simulink model "system_model_NMPC"  (R2025b)
settings: Solver=ode45  StartTime=0.0  StopTime=40000  MaxStep=1.5  RelTol=1e-9
values from neighbouring files (symbols this model uses):
  a_leader = 6786 *10^3    (= 6786000)    [main_setup.m]
  delta_a_ref = 0    [ControllerPerformance.m]    (also in evaluate_orbit_control.m = expandReference(delta_a_ref, n, 'delta_a_ref'); main_setup.m)
  delta_lambda_ref = 20/a_leader    [ControllerPerformance.m]    (also in evaluate_orbit_control.m = expandReference(delta_lambda_ref, n, 'delta_lambda_ref'); main_setup.m = 2.94724432655e-06)
  earth_radi = 6371*10^3    (= 6371000)    [main_setup.m]
  J2 = 1.08263e-3    (= 0.00108263)    [nmpc_orbit_state.m]
  J_2 = 1.08263 * 10^(-3)    (= 0.00108263)    [main_setup.m]
  Kd_follower = 2*zeta_follower*wn_follower *                [Jx_follower ... (first row only)    [ATTITUDE_INITIALS.m]
  Kd_leader = 2*zeta_leader*wn_leader *              [Jx_leader ... (first row only)    [ATTITUDE_INITIALS.m]
  Kp_follower = [Jx_follower ... (first row only)    [ATTITUDE_INITIALS.m]
  Kp_leader = [Jx_leader ... (first row only)    [ATTITUDE_INITIALS.m]
  m_f = 2    [main_setup.m]
  m_l = 2    [main_setup.m]
  Mmax_follower = [3.2e-3 ... (first row only)    [ATTITUDE_INITIALS.m]
  Mmax_leader = [3.2e-3 ... (first row only)    [ATTITUDE_INITIALS.m]
  mu = G*earth_mass    (= 398589196000000)    [main_setup.m]    (also in nmpc_orbit_state.m)
  rho_leader = mean_rho_500km    (= 7.3e-13)    [main_setup.m]
undefined symbols (not defined in the file or in its folder): beta0_sdre, beta_max_sdre, beta_min_sdre, Q_sdre, R_sdre
libraries: mpclib x1
(part 1 of 3)
settings Model: Creator=andrefan  LastModifiedBy=Lenovo
settings DataIOCC: FinalStateName=system_modelSimState  InitialState=system_modelSimState  SaveFinalState=on  SaveOperatingPoint=on
settings OptimizationCC: DefaultParameterBehavior=Inlined  UseDivisionForNetSlopeComputation=on  GainParamInheritBuiltInType=on  UseFloatMulNetSlope=on  InlineInvariantSignals=on  FunctionInliningControlUserFunctions=Never  FunctionInliningControlMWFunctions=Readability  FunctionInliningControlMWUserFunctions=Never  PassReuseOutputArgsAs=Individual arguments  ZeroExternalMemoryAtStartup=off  ZeroInternalMemoryAtStartup=off  NoFixptDivByZeroProtection=on  EfficientFloat2IntCast=on  LifeSpan=1  OptimizeBlockOrder=speed  DifferentSizesBufferReuse=on  EfficientTunableParamExpr=on
settings DebuggingCC: ParameterTunabilityLossMsg=error
settings HardwareCC: ProdLongLongMode=on
settings SFSimCC: MATLABDynamicMemAlloc=off
settings RTWCC: SystemTargetFile=ert.tlc  GenCodeOnly=on  TemplateMakefile=ert_default_tmf  BuildConfiguration=Debug  GPUComputeCapability=3.5  Description=Embedded Coder
settings CodeAppCC: ForceParamTrailComments=on  IgnoreCustomStorageClasses=off  OperatorAnnotations=on  SimulinkDataObjDesc=on  SFDataObjDesc=on  CustomSymbolStrGlobalVar=rt$N$M  CustomSymbolStrType=$N$M  CustomSymbolStrFcn=$N$M$F  CustomSymbolStrMacro=$N$M  InsertBlockDesc=on
settings ERTTargetCC: ERTCustomFileTemplate=example_file_process.tlc  ERTFilePackagingFormat=CompactWithDataFile  TargetLangStandard=C99 (ISO)  GenerateSampleERTMain=on  IncludeMdlTerminateFcn=off  CombineSignalStateStructs=on  SupportAbsoluteTime=off  SupportComplex=off  SupportContinuousTime=on  SupportNonInlinedSFcns=on

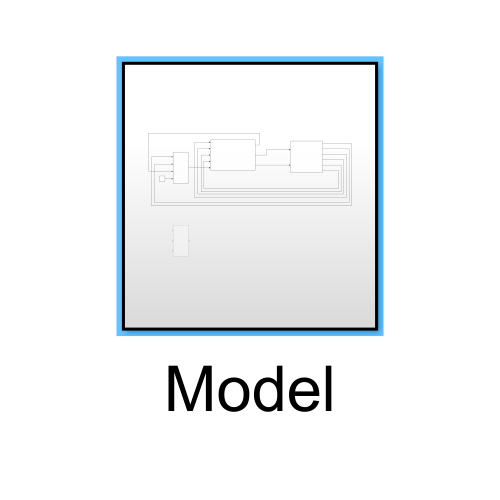
[thumbnail: Simulink's stored preview of the top-level diagram]
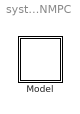
== system system_model_NMPC ==
  Model : Subsystem

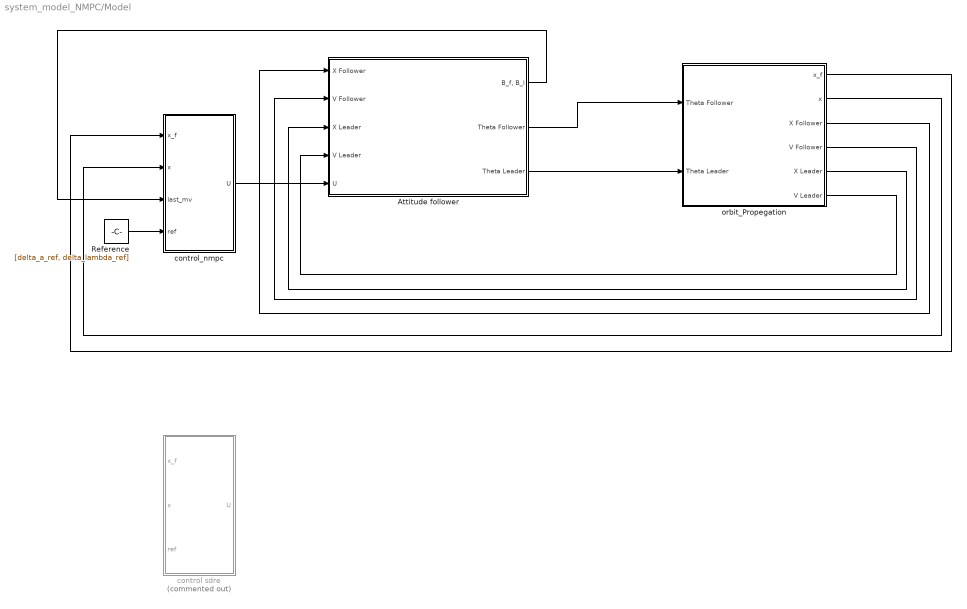
== system system_model_NMPC/Model ==
  "Attitude follower " : Subsystem
  Reference : Constant  Value=[delta_a_ref, delta_lambda_ref]
  control sdre : Subsystem  Commented=on
  control_nmpc : Subsystem
  orbit_Propegation : Subsystem
  wires:
  orbit_Propegation/1(x_f) -> control_nmpc/1(x_f)
  orbit_Propegation/2(x) -> control_nmpc/2(x)
  Reference/1 -> control_nmpc/4(ref)
  orbit_Propegation/3(X Follower) -> "Attitude follower "/1(X Follower)
  orbit_Propegation/4(V Follower) -> "Attitude follower "/2(V Follower)
  orbit_Propegation/5(X Leader) -> "Attitude follower "/3(X Leader)
  orbit_Propegation/6(V Leader) -> "Attitude follower "/4(V Leader)
  "Attitude follower "/2(Theta Follower) -> orbit_Propegation/1(Theta Follower)
  "Attitude follower "/3(Theta Leader) -> orbit_Propegation/2(Theta Leader)
  control_nmpc/1(U) -> "Attitude follower "/5(U)
  "Attitude follower "/1("B_f, B_l") -> control_nmpc/3(last_mv)

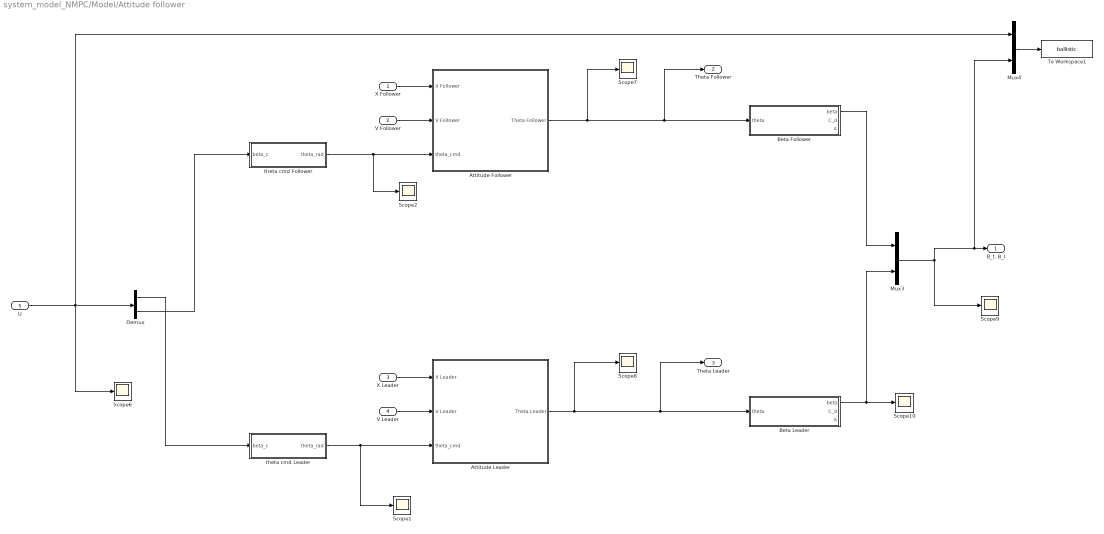
== system system_model_NMPC/Model/Attitude follower  ==
  X Follower : Inport
  V Follower : Inport  Port=2
  X Leader : Inport  Port=3
  V Leader : Inport  Port=4
  U : Inport  Port=5
  Attitude Follower : Subsystem
  Attitude Leader : Subsystem
  Beta Follower : MATLAB Function  TreatAsAtomicUnit=on
  Beta Leader : MATLAB Function  TreatAsAtomicUnit=on
  Demux : Demux  Outputs=2
  Mux3 : Mux  Inputs=2
  Mux4 : Mux  Inputs=2
  Scope{1..2,6..10} (7 alike) : Scope
      Scope1 settings: ActiveDisplayYMinimum=-0.045913062602693733  ActiveDisplayYMaximum=1.4555864748650962  DataLoggingVariableName=ScopeData43
      Scope10 settings: ActiveDisplayYMinimum=-0.0089508661365174519  ActiveDisplayYMaximum=0.27107619634307356  DataLoggingVariableName=ScopeData40
      Scope2 settings: ActiveDisplayYMinimum=-0.18250820694100406  ActiveDisplayYMaximum=1.6425738624690367
      Scope6 settings: ActiveDisplayYMinimum=0.0048104776645491263  ActiveDisplayYMaximum=0.08683060912495788  DataLoggingVariableName=ScopeData41
      Scope7 settings: ActiveDisplayYMinimum=-0.14955674609276967  ActiveDisplayYMaximum=1.3420939307289279  DataLoggingVariableName=ScopeData42
      Scope8 settings: ActiveDisplayYMinimum=-4.5513250658678969E-5  ActiveDisplayYMaximum=0.0004096192559281108  DataLoggingVariableName=ScopeData43
      Scope9 settings: ActiveDisplayYMinimum=-0.051056264121872613  ActiveDisplayYMaximum=0.257673572261877  DataLoggingVariableName=ScopeData38
  To Workspace1 : ToWorkspace  VariableName=ballistic  SaveFormat=Timeseries  SampleTime=-1
  theta cmd Follower : MATLAB Function  TreatAsAtomicUnit=on
  theta cmd Leader : MATLAB Function  TreatAsAtomicUnit=on
  "B_f, B_l" : Outport
  Theta Follower : Outport  Port=2
  Theta Leader : Outport  Port=3
  wires:
  X Follower/1 -> Attitude Follower/1(X Follower)
  V Follower/1 -> Attitude Follower/2(V Follower)
  X Leader/1 -> Attitude Leader/1(X Leader)
  V Leader/1 -> Attitude Leader/2(V Leader)
  theta cmd Leader/1(theta_rad) -> Scope1/1, Attitude Leader/3(theta_cmd)
  theta cmd Follower/1(theta_rad) -> Scope2/1, Attitude Follower/3(theta_cmd)
  Attitude Follower/1(Theta Follower) -> Theta Follower/1, Beta Follower/1(theta), Scope7/1
  Attitude Leader/1(Theta Leader) -> Scope8/1, Theta Leader/1, Beta Leader/1(theta)
  Beta Leader/1(beta) -> Mux3/2, Scope10/1
  Mux3/1 -> Scope9/1, Mux4/2, "B_f, B_l"/1
  Beta Follower/1(beta) -> Mux3/1
  Mux4/1 -> To Workspace1/1
  U/1 -> Mux4/1, Scope6/1, Demux/1
  Demux/1 -> theta cmd Leader/1(beta_c)
  Demux/2 -> theta cmd Follower/1(beta_c)

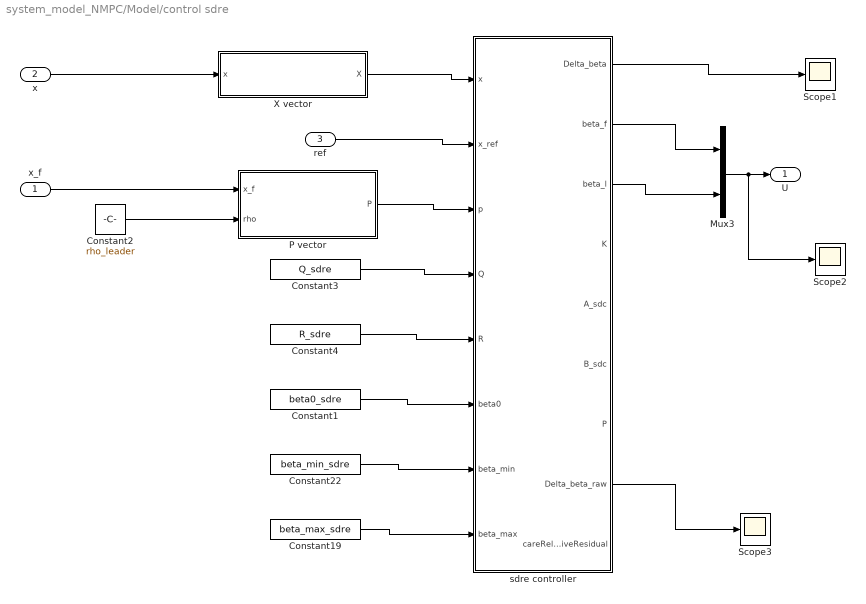
== system system_model_NMPC/Model/control sdre ==
  x_f : Inport
  x : Inport  Port=2
  ref : Inport  Port=3
  Constant1 : Constant  Value=beta0_sdre
  Constant19 : Constant  Value=beta_max_sdre
  Constant2 : Constant  Value=rho_leader
  Constant22 : Constant  Value=beta_min_sdre
  Constant3 : Constant  Value=Q_sdre
  Constant4 : Constant  Value=R_sdre
  Mux3 : Mux  Inputs=2
  P vector : MATLAB Function  TreatAsAtomicUnit=on
  Scope1 : Scope
      settings: ActiveDisplayYMinimum=-0.0032921639354863029  ActiveDisplayYMaximum=-0.0014749131731903909  DataLoggingVariableName=ScopeData14
  Scope2 : Scope
      settings: ActiveDisplayYMinimum=0.0407755493500229  ActiveDisplayYMaximum=0.054229976864297966  DataLoggingVariableName=ScopeData3
  Scope3 : Scope
      settings: ActiveDisplayYMinimum=0.033685370004966811  ActiveDisplayYMaximum=0.084038625678476891  DataLoggingVariableName=ScopeData5
  X vector : MATLAB Function  TreatAsAtomicUnit=on
  sdre controller : MATLAB Function  TreatAsAtomicUnit=on
  U : Outport
  wires:
  P vector/1(P) -> sdre controller/3(p)
  Constant2/1 -> P vector/2(rho)
  x_f/1 -> P vector/1(x_f)
  x/1 -> X vector/1(x)
  X vector/1(X) -> sdre controller/1(x)
  Constant19/1 -> sdre controller/8(beta_max)
  Constant22/1 -> sdre controller/7(beta_min)
  Constant1/1 -> sdre controller/6(beta0)
  Constant3/1 -> sdre controller/4(Q)
  sdre controller/2(beta_f) -> Mux3/1
  sdre controller/3(beta_l) -> Mux3/2
  Mux3/1 -> U/1, Scope2/1
  ref/1 -> sdre controller/2(x_ref)
  sdre controller/1(Delta_beta) -> Scope1/1
  sdre controller/8(Delta_beta_raw) -> Scope3/1
  Constant4/1 -> sdre controller/5(R)

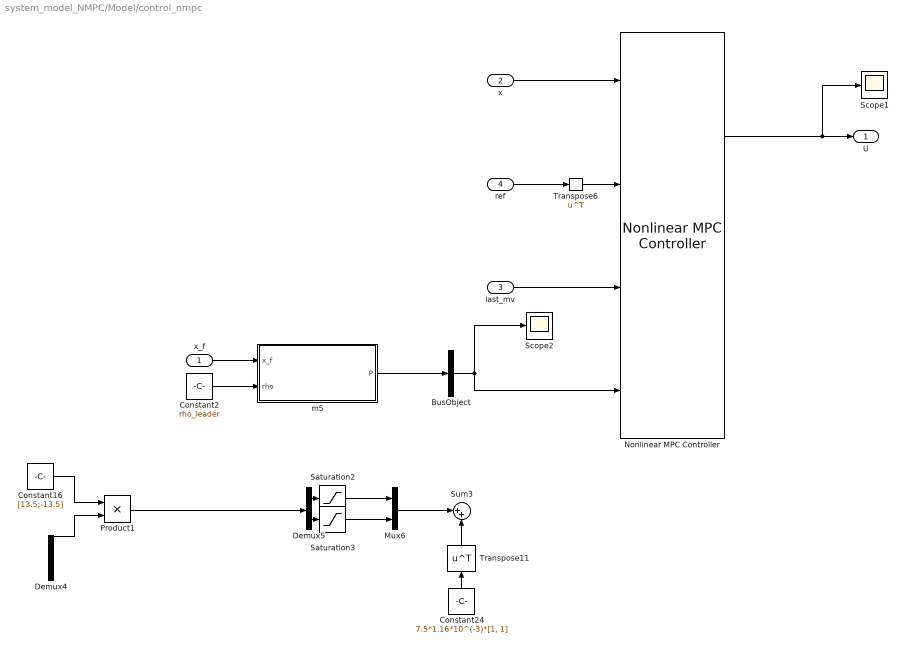
== system system_model_NMPC/Model/control_nmpc ==
  x_f : Inport
  x : Inport  Port=2
  last_mv : Inport  Port=3
  ref : Inport  Port=4
  BusObject : BusCreator  Inputs=1  OutDataTypeStr=Bus: BusObject  NonVirtualBus=on
      settings: InheritFromInputs=off
  Constant16 : Constant  Value=[13.5;-13.5]
  Constant2 : Constant  Value=rho_leader
  Constant24 : Constant  Value=7.5*1.16*10^(-3)*[1, 1]
  Demux4 : Demux  Outputs=6
  Demux5 : Demux  Outputs=2
  Mux6 : Mux  Inputs=2
  Nonlinear MPC Controller : mpclib/Nonlinear MPC Controller  nlmpcobj=nlobj  UseObjectTs=on  TsControl=20  UseMEX=off  md_enabled=off  mvtarget_enabled=off  param_enabled=on  cost_enabled=on  mvseq_enabled=off  stateseq_enabled=off  ovseq_enabled=off  slack_enabled=off  status_enabled=off  ov_min=off  ov_max=off  mv_min=off  mv_max=off  mvrate_min=off  mvrate_max=off  state_min=off  state_max=off  ov_weight=off  mv_weight=off  mvrate_weight=off  ecr_weight=off  nlp_initialize=off
  Product1 : Product
  Saturation2 : Saturate  UpperLimit=inf  LowerLimit=0.000348
  Saturation3 : Saturate  UpperLimit=inf  LowerLimit=0.000348
  Scope1 : Scope
      settings: ActiveDisplayYMinimum=0.00481047337988073  ActiveDisplayYMaximum=0.086830624071647655  DataLoggingVariableName=ScopeData14
  Scope2 : Scope
      settings: ActiveDisplayYMinimum=-9.0946582247123644E+6  ActiveDisplayYMaximum=2.6536439957668819E+7  DataLoggingVariableName=ScopeData35
  Sum3 : Sum  Inputs=|++
  Transpose11 : Math  Operator=transpose
  Transpose6 : Math  Operator=transpose
  m5 : MATLAB Function  TreatAsAtomicUnit=on
  U : Outport
  wires:
  m5/1(P) -> BusObject/1
  Transpose6/1 -> Nonlinear MPC Controller/2
  x/1 -> Nonlinear MPC Controller/1
  ref/1 -> Transpose6/1
  x_f/1 -> m5/1(x_f)
  last_mv/1 -> Nonlinear MPC Controller/3
  Constant2/1 -> m5/2(rho)
  BusObject/1 -> Scope2/1, Nonlinear MPC Controller/4
  Nonlinear MPC Controller/1 -> Scope1/1, U/1
  Demux5/1 -> Saturation2/1
  Mux6/1 -> Sum3/1
  Transpose11/1 -> Sum3/2
  Saturation3/1 -> Mux6/2
  Product1/1 -> Demux5/1
  Constant16/1 -> Product1/1
  Saturation2/1 -> Mux6/1
  Constant24/1 -> Transpose11/1
  Demux4/1 -> Product1/2
  Demux5/2 -> Saturation3/1

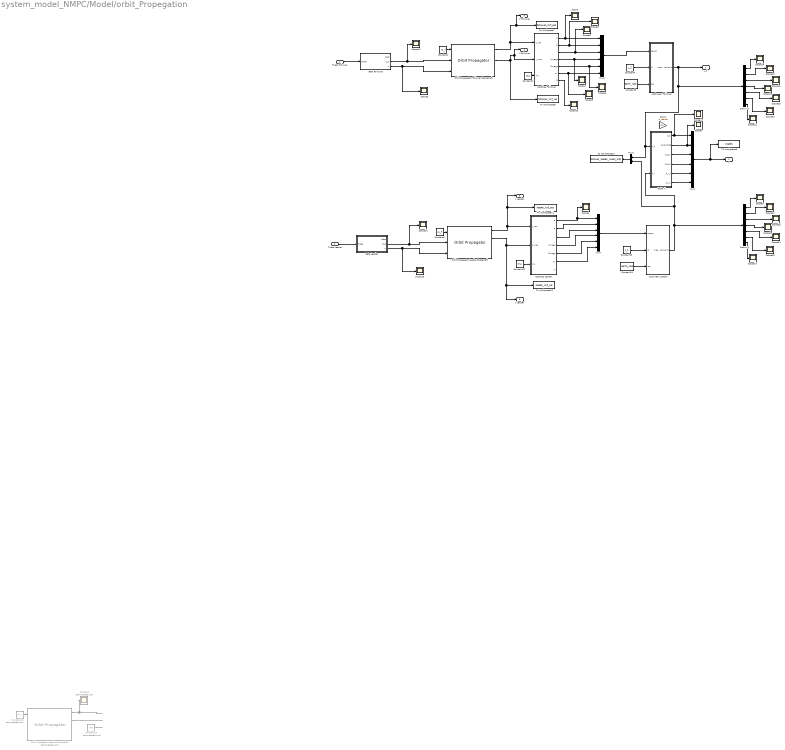
== system system_model_NMPC/Model/orbit_Propegation ==
  Theta Follower : Inport
  Theta Leader : Inport  Port=2
  Beta Follower : MATLAB Function  TreatAsAtomicUnit=on
  Beta Leader : MATLAB Function  TreatAsAtomicUnit=on
  Cart2kep Follower : MATLAB Function  TreatAsAtomicUnit=on
  Cart2kep Leader : MATLAB Function  TreatAsAtomicUnit=on
  Constant1 : Constant  Value=m_f
  Constant12 : Constant  Value=mu
  Constant13 : Constant  Value=J_2
  Constant14 : Constant  Value=earth_radi
  Constant18 : Constant  Commented=on  Value=m_l
  Constant19 : Constant  Commented=on  Value=mu
  Constant2 : Constant  Value=mu
  Constant4 : Constant  Value=J_2
  Constant5 : Constant  Value=earth_radi
  Constant6 : Constant  Value=m_f
  Delta X : MATLAB Function  TreatAsAtomicUnit=on
  Demux1 : Demux  Outputs=7
  Demux2 : Demux  Outputs=7
  Gain2 : Gain  Gain=a_leader
  Mux1 : Mux  Inputs=6
  Mux6 : Mux  Inputs=6
  Mux7 : Mux  Inputs=6
  Mux9 : Mux  Inputs=2
  Orbit Propagator Follower Spacecraft : OrbitPropagator  propagator=Numerical (high precision)  massSrc=Port  mass=2.0  semiMajorAxis=a_follower  eccentricity=e_follower  inclination=i_follower  raan=Omega_follower  argPeriapsis=omega_follower  trueAnomaly=TA_follower  inertialPosition=[3649700.0 3308200.0 -4676600.0]  inertialVelocity=[-2750.8 6666.4 2573.4]  fixedPosition=[-4142689.0 -2676864.7 -4669861.6]  fixedVelocity=[1452.7 -6720.7 2568.1]  gravityModel=Oblate ellipsoid (J2)  customR=3396200  customMu=4.305e13  customJ2=1.0826269e-03  customOmega=4.06125949e-3  useDrag=on  useOxygen=off  dragCoeffSrc=Port  dragCoeff=2.3  dragAreaSrc=Port  dragArea=0.6  useThirdBodyGravity=on
  Orbit Propagator Leader Spacecraft : OrbitPropagator  propagator=Numerical (high precision)  massSrc=Port  mass=2.0  semiMajorAxis=a_leader  eccentricity=e_leader  inclination=i_leader  raan=Omega_leader  argPeriapsis=omega_leader  trueAnomaly=TA_leader  inertialPosition=[3649700.0 3308200.0 -4676600.0]  inertialVelocity=[-2750.8 6666.4 2573.4]  fixedPosition=[-4142689.0 -2676864.7 -4669861.6]  fixedVelocity=[1452.7 -6720.7 2568.1]  gravityModel=Oblate ellipsoid (J2)  customR=3396200  customMu=4.305e13  customJ2=1.0826269e-03  customOmega=4.06125949e-3  outputTransform=on  useDrag=on  useOxygen=off  dragCoeffSrc=Port  dragCoeff=2.3  dragAreaSrc=Port  dragArea=0.6  useThirdBodyGravity=on
  Orbit Propagator Leader Spacecraft1 : OrbitPropagator  Commented=on  propagator=Numerical (high precision)  massSrc=Port  mass=2.0  stateFormatNum=ICRF state vector  inclination=20  argPeriapsis=0  trueAnomaly=100.001  inertialPosition=[(6371+500)*10^3 0 0]  inertialVelocity=[0 7.616*10^3 0]  fixedPosition=[-4142689.0 -2676864.7 -4669861.6]  fixedVelocity=[1452.7 -6720.7 2568.1]  gravityModel=Oblate ellipsoid (J2)  customR=3396200  customMu=4.305e13  customJ2=1.0826269e-03  customOmega=4.06125949e-3  outputTransform=on  useDrag=on  useOxygen=off  dragCoeffSrc=Port  dragCoeff=2.3  dragAreaSrc=Port  dragArea=0.6  useThirdBodyGravity=on
  Scope{,1..27} (28 alike) : Scope
      Scope settings: ActiveDisplayYMinimum=6.7851539643780729E+6  ActiveDisplayYMaximum=6.7880499452324249E+6  DataLoggingVariableName=ScopeData10
      Scope1 settings: ActiveDisplayYMinimum=-1  ActiveDisplayYMaximum=1  DataLoggingVariableName=ScopeData17
      Scope10 settings: ActiveDisplayYMinimum=-0.38136764312903559  ActiveDisplayYMaximum=6.0798469595030005  DataLoggingVariableName=ScopeData18
      Scope11 settings: ActiveDisplayYMinimum=2.2815669907857319  ActiveDisplayYMaximum=2.6381571811562821  DataLoggingVariableName=ScopeData34
      Scope12 settings: ActiveDisplayYMinimum=-0.38136764312903559  ActiveDisplayYMaximum=6.0798469595030005  DataLoggingVariableName=ScopeData36
      Scope13 settings: ActiveDisplayYMinimum=-0.0027186651405793072  ActiveDisplayYMaximum=0.12936498566288834  DataLoggingVariableName=ScopeData37
      Scope14 settings: ActiveDisplayYMinimum=6.7865902805892117E+6  ActiveDisplayYMaximum=6.78661319696359E+6  DataLoggingVariableName=ScopeData6
      Scope15 settings: ActiveDisplayYMinimum=0.011257756358800488  ActiveDisplayYMaximum=0.011347804883761338  DataLoggingVariableName=ScopeData7
      Scope16 settings: ActiveDisplayYMinimum=6.786569104627762E+6  ActiveDisplayYMaximum=6.7866627861652E+6  DataLoggingVariableName=ScopeData8
      Scope17 settings: ActiveDisplayYMinimum=-3.0771886432165871E-6  ActiveDisplayYMaximum=1.6457538924105332E-6  DataLoggingVariableName=ScopeData19
      Scope18 settings: ActiveDisplayYMinimum=6.786569104627762E+6  ActiveDisplayYMaximum=6.7866627861652E+6  DataLoggingVariableName=ScopeData9
      Scope19 settings: ActiveDisplayYMinimum=6.786569104627762E+6  ActiveDisplayYMaximum=6.7866627861652E+6  DataLoggingVariableName=ScopeData11
      Scope2 settings: ActiveDisplayYMinimum=0.0036465468505335538  ActiveDisplayYMaximum=0.067181078345198028  DataLoggingVariableName=ScopeData33
      Scope20 settings: ActiveDisplayYMinimum=6.786569104627762E+6  ActiveDisplayYMaximum=6.7866627861652E+6  DataLoggingVariableName=ScopeData12
      Scope21 settings: ActiveDisplayYMinimum=6.786569104627762E+6  ActiveDisplayYMaximum=6.7866627861652E+6  DataLoggingVariableName=ScopeData13
      Scope22 settings: ActiveDisplayYMinimum=0.011259402063854809  ActiveDisplayYMaximum=0.01134830549609502  DataLoggingVariableName=ScopeData15
      Scope23 settings: ActiveDisplayYMinimum=0.34914544683083076  ActiveDisplayYMaximum=0.349147724859292  DataLoggingVariableName=ScopeData16
      Scope24 settings: ActiveDisplayYMinimum=1.6484577890542687  ActiveDisplayYMaximum=1.6598721225746775  DataLoggingVariableName=ScopeData20
      Scope25 settings: ActiveDisplayYMinimum=0.32273994775939485  ActiveDisplayYMaximum=0.34925286311678672  DataLoggingVariableName=ScopeData23
      Scope26 settings: ActiveDisplayYMinimum=-0.78411859721448307  ActiveDisplayYMaximum=7.06771246867728  DataLoggingVariableName=ScopeData39
      Scope27 settings: ActiveDisplayYMinimum=-0.7840920546033614  ActiveDisplayYMaximum=7.0676944011099723  DataLoggingVariableName=ScopeData44
      Scope3 settings: ActiveDisplayYMinimum=6.7866086263097124E+6  ActiveDisplayYMaximum=6.7866453783500874E+6  DataLoggingVariableName=ScopeData45
      Scope4 settings: ActiveDisplayYMinimum=-2.9851895780546657E-6  ActiveDisplayYMaximum=1.8401517445560543E-5  DataLoggingVariableName=ScopeData21
      Scope5 settings: ActiveDisplayYMinimum=-5.3552746938434178E-5  ActiveDisplayYMaximum=0.00328678328931705  DataLoggingVariableName=ScopeData22
      Scope6 settings: ActiveDisplayYMinimum=-1  ActiveDisplayYMaximum=1  DataLoggingVariableName=ScopeData24
      Scope7 settings: ActiveDisplayYMinimum=-0.6787796137699198  ActiveDisplayYMaximum=7.5670809371302168  DataLoggingVariableName=ScopeData25
      Scope8 settings: ActiveDisplayYMinimum=0.34236884466589917  ActiveDisplayYMaximum=0.35312198954443319  DataLoggingVariableName=ScopeData27
      Scope9 settings: ActiveDisplayYMinimum=-0.78522346169078239  ActiveDisplayYMaximum=7.0676517910578136  DataLoggingVariableName=ScopeData32
  Scope38 : Scope  Commented=on
      settings: ActiveDisplayYMinimum=-858875.74756  ActiveDisplayYMaximum=7.72987508306E+6  DataLoggingVariableName=ScopeData4
  To Workspace10 : ToWorkspace  VariableName=follower_leader_mean_orbi  SaveFormat=Timeseries  SampleTime=-1
  To Workspace11 : ToWorkspace  VariableName=leader_icrf_pos  SaveFormat=Timeseries  SampleTime=-1
  To Workspace12 : ToWorkspace  VariableName=leader_icrf_vel  SaveFormat=Timeseries  SampleTime=-1
  To Workspace7 : ToWorkspace  VariableName=follower_icrf_pos  SaveFormat=Timeseries  SampleTime=-1
  To Workspace8 : ToWorkspace  VariableName=follower_icrf_vel  SaveFormat=Timeseries  SampleTime=-1
  To Workspace9 : ToWorkspace  VariableName=states  SaveFormat=Timeseries  SampleTime=-1
  osc2mean Follower : MATLAB Function  TreatAsAtomicUnit=on
  osc2mean Leader : MATLAB Function  TreatAsAtomicUnit=on
  x_f : Outport
  x : Outport  Port=2
  X Follower : Outport  Port=3
  V Follower : Outport  Port=4
  X Leader : Outport  Port=5
  V Leader : Outport  Port=6
  wires:
  Orbit Propagator Leader Spacecraft1/1 -> Scope38/1
  Constant18/1 -> Orbit Propagator Leader Spacecraft1/1
  Orbit Propagator Leader Spacecraft1/2 -> ?
  Constant19/1 -> ?
  Cart2kep Follower/1(a) -> Scope/1, Mux6/1
  Constant2/1 -> Cart2kep Follower/3(mu)
  Mux1/1 -> x/1, To Workspace9/1
  Cart2kep Follower/2(e) -> Scope5/1, Mux6/2
  Orbit Propagator Follower Spacecraft/2 -> V Follower/1, Cart2kep Follower/2(v_vec), To Workspace8/1
  Constant6/1 -> Orbit Propagator Leader Spacecraft/1
  Constant1/1 -> Orbit Propagator Follower Spacecraft/1
  Cart2kep Leader/1(a) -> Scope1/1, Mux7/1
  Delta X/6(d_i_y) -> Mux1/6
  Theta Leader/1 -> Beta Leader/1(theta)
  Cart2kep Follower/5(Omega) -> Mux6/5, Scope6/1
  Cart2kep Leader/4(omega) -> Mux7/4
  Mux7/1 -> osc2mean Leader/1(oeosc)
  Cart2kep Leader/2(e) -> Mux7/2
  Beta Leader/3(A) -> Scope13/1, Orbit Propagator Leader Spacecraft/3
  Cart2kep Leader/5(Omega) -> Mux7/5
  Cart2kep Leader/6(nu) -> Mux7/6
  Delta X/5(d_i_x) -> Mux1/5
  Constant12/1 -> Cart2kep Leader/3(mu)
  Delta X/4(d_e_y) -> Mux1/4
  Orbit Propagator Leader Spacecraft/1 -> X Leader/1, To Workspace11/1, Cart2kep Leader/1(r_vec)
  Beta Follower/2(C_d) -> Scope11/1, Orbit Propagator Follower Spacecraft/2
  Beta Follower/3(A) -> Scope2/1, Orbit Propagator Follower Spacecraft/3
  Constant5/1 -> osc2mean Follower/3(req)
  Constant14/1 -> osc2mean Leader/3(req)
  Delta X/1(d_a) -> Mux1/1, Scope17/1
  Cart2kep Follower/4(omega) -> Scope7/1, Mux6/4
  Cart2kep Follower/6(nu) -> Mux6/6, Scope9/1
  Orbit Propagator Leader Spacecraft/2 -> V Leader/1, To Workspace12/1, Cart2kep Leader/2(v_vec)
  Constant13/1 -> osc2mean Leader/2(j2)
  Delta X/2(d_lambda) -> Mux1/2, Scope4/1
  Orbit Propagator Follower Spacecraft/1 -> X Follower/1, To Workspace7/1, Cart2kep Follower/1(r_vec)
  Cart2kep Follower/3(i) -> Scope8/1, Mux6/3
  Delta X/3(d_e_x) -> Mux1/3
  Beta Leader/2(C_d) -> Scope12/1, Orbit Propagator Leader Spacecraft/2
  Theta Follower/1 -> Beta Follower/1(theta)
  Cart2kep Leader/3(i) -> Mux7/3
  Mux9/1 -> To Workspace10/1
  Cart2kep Follower/7(M) -> Scope10/1
  Constant4/1 -> osc2mean Follower/2(j2)
  Mux6/1 -> osc2mean Follower/1(oeosc)
  osc2mean Follower/1(mean_elements) -> x_f/1, Mux9/1, Delta X/1(x_f), Demux2/1
  Demux2/1 -> Scope14/1
  Demux2/2 -> Scope15/1
  Demux2/3 -> Scope16/1
  Demux2/5 -> Scope18/1
  Demux2/4 -> Scope19/1
  Demux2/6 -> Scope20/1
  Demux2/7 -> Scope21/1
  Demux1/2 -> Scope22/1
  Demux1/6 -> Scope26/1
  osc2mean Leader/1(mean_elements) -> Demux1/1, Mux9/2, Delta X/2(x_l)
  Demux1/7 -> Scope27/1
  Demux1/4 -> Scope25/1
  Demux1/1 -> Scope3/1
  Demux1/5 -> Scope24/1
  Demux1/3 -> Scope23/1

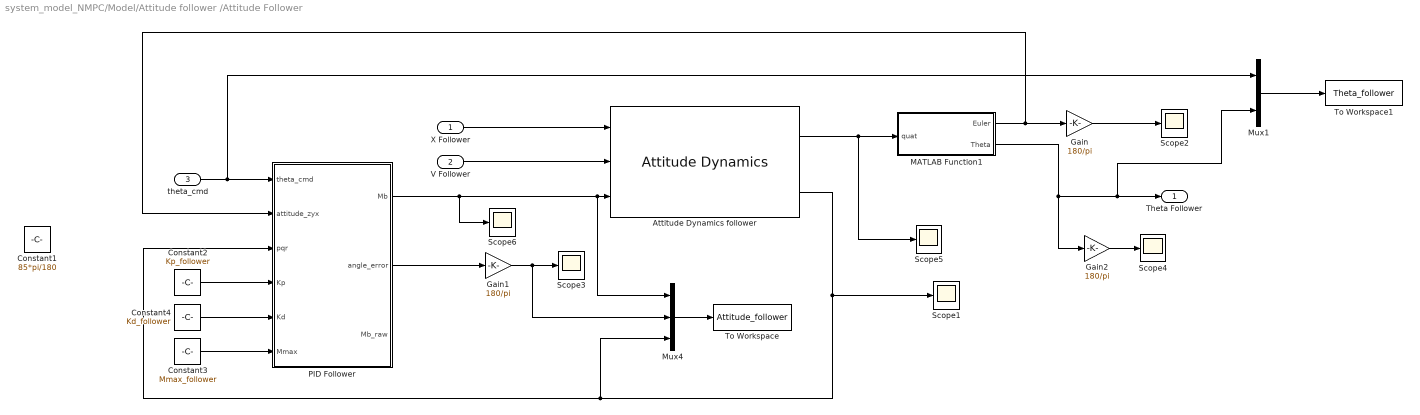
== system system_model_NMPC/Model/Attitude follower /Attitude Follower ==
  X Follower : Inport
  V Follower : Inport  Port=2
  theta_cmd : Inport  Port=3
  Attitude Dynamics follower : AttitudeDynamics  dateOut=off  action=Error  mass=m_sat_follower  inertia=J_follower  attitudeFrame=LVLH  attitude=q0_follower  attitudeRate=omega0_follower  useGravGrad=off  angleUnits=Radians
  Constant1 : Constant  Value=85*pi/180
  Constant2 : Constant  Value=Kp_follower
  Constant3 : Constant  Value=Mmax_follower
  Constant4 : Constant  Value=Kd_follower
  Gain : Gain  Gain=180/pi
  Gain1 : Gain  Gain=180/pi
  Gain2 : Gain  Gain=180/pi
  MATLAB Function1 : MATLAB Function  TreatAsAtomicUnit=on
  Mux1 : Mux  Inputs=2
  Mux4 : Mux  Inputs=3
  PID Follower : MATLAB Function  TreatAsAtomicUnit=on
  Scope{1..6} (6 alike) : Scope
      Scope1 settings: ActiveDisplayYMinimum=-0.0067898026228066909  ActiveDisplayYMaximum=0.0069957960553773384  DataLoggingVariableName=ScopeData28
      Scope2 settings: ActiveDisplayYMinimum=-10.533126247503391  ActiveDisplayYMaximum=94.370566087990781  DataLoggingVariableName=ScopeData29
      Scope3 settings: ActiveDisplayYMinimum=-17.088160840258741  ActiveDisplayYMaximum=17.56795566474937  DataLoggingVariableName=ScopeData30
      Scope4 settings: ActiveDisplayYMinimum=-23.696067658896066  ActiveDisplayYMaximum=96.143567971393608  DataLoggingVariableName=ScopeData31
      Scope5 settings: ActiveDisplayYMinimum=-3.1008685090601471  ActiveDisplayYMaximum=2.0444369747055768  DataLoggingVariableName=ScopeData26
      Scope6 settings: ActiveDisplayYMinimum=-2.2085384193141472E-7  ActiveDisplayYMaximum=7.0192334116134588E-8
  To Workspace : ToWorkspace  VariableName=Attitude_follower  SaveFormat=Timeseries  SampleTime=-1
  To Workspace1 : ToWorkspace  VariableName=Theta_follower  SaveFormat=Timeseries  SampleTime=-1
  Theta Follower : Outport
  wires:
  Attitude Dynamics follower/1 -> Scope5/1, MATLAB Function1/1(quat)
  V Follower/1 -> Attitude Dynamics follower/2
  Constant3/1 -> PID Follower/6(Mmax)
  X Follower/1 -> Attitude Dynamics follower/1
  Attitude Dynamics follower/2 -> Mux4/3, PID Follower/3(pqr), Scope1/1
  MATLAB Function1/1(Euler) -> PID Follower/2(attitude_zyx), Gain/1
  Constant2/1 -> PID Follower/4(Kp)
  Constant4/1 -> PID Follower/5(Kd)
  Gain/1 -> Scope2/1
  PID Follower/2(angle_error) -> Gain1/1
  Gain1/1 -> Mux4/2, Scope3/1
  MATLAB Function1/2(Theta) -> Gain2/1, Mux1/2, Theta Follower/1
  Gain2/1 -> Scope4/1
  theta_cmd/1 -> Mux1/1, PID Follower/1(theta_cmd)
  PID Follower/1(Mb) -> Scope6/1, Mux4/1, Attitude Dynamics follower/3
  Mux4/1 -> To Workspace/1
  Mux1/1 -> To Workspace1/1

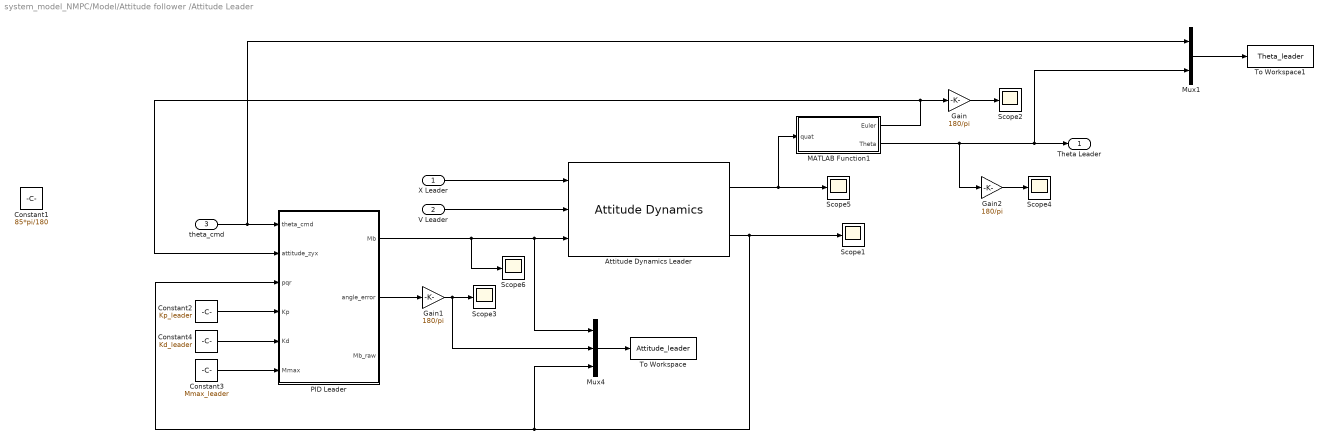
== system system_model_NMPC/Model/Attitude follower /Attitude Leader ==
  X Leader : Inport
  V Leader : Inport  Port=2
  theta_cmd : Inport  Port=3
  Attitude Dynamics Leader : AttitudeDynamics  dateOut=off  action=Error  mass=m_sat_leader  inertia=J_leader  attitudeFrame=LVLH  attitude=q0_leader  attitudeRate=omega0_leader  useGravGrad=off  angleUnits=Radians
  Constant1 : Constant  Value=85*pi/180
  Constant2 : Constant  Value=Kp_leader
  Constant3 : Constant  Value=Mmax_leader
  Constant4 : Constant  Value=Kd_leader
  Gain : Gain  Gain=180/pi
  Gain1 : Gain  Gain=180/pi
  Gain2 : Gain  Gain=180/pi
  MATLAB Function1 : MATLAB Function  TreatAsAtomicUnit=on
  Mux1 : Mux  Inputs=2
  Mux4 : Mux  Inputs=3
  PID Leader : MATLAB Function  TreatAsAtomicUnit=on
  Scope{1..6} (6 alike) : Scope
      Scope1 settings: ActiveDisplayYMinimum=-0.53072756087043993  ActiveDisplayYMaximum=1.099418115704675  DataLoggingVariableName=ScopeData28
      Scope2 settings: ActiveDisplayYMinimum=-260.43791746613203  ActiveDisplayYMaximum=260.493332499561  DataLoggingVariableName=ScopeData29
      Scope3 settings: ActiveDisplayYMinimum=-96.882096317677025  ActiveDisplayYMaximum=35.382868121511578  DataLoggingVariableName=ScopeData30
      Scope4 settings: ActiveDisplayYMinimum=-10.618129191017523  ActiveDisplayYMaximum=95.563162719157731  DataLoggingVariableName=ScopeData31
      Scope5 settings: ActiveDisplayYMinimum=-3.1008685090601471  ActiveDisplayYMaximum=2.0444369747055768  DataLoggingVariableName=ScopeData26
      Scope6 settings: ActiveDisplayYMinimum=-6.1878545082380226E-5  ActiveDisplayYMaximum=0.0002169496404154156  DataLoggingVariableName=ScopeData2
  To Workspace : ToWorkspace  VariableName=Attitude_leader  SaveFormat=Timeseries  SampleTime=-1
  To Workspace1 : ToWorkspace  VariableName=Theta_leader  SaveFormat=Timeseries  SampleTime=-1
  Theta Leader : Outport
  wires:
  Attitude Dynamics Leader/1 -> MATLAB Function1/1(quat), Scope5/1
  V Leader/1 -> Attitude Dynamics Leader/2
  Constant3/1 -> PID Leader/6(Mmax)
  X Leader/1 -> Attitude Dynamics Leader/1
  MATLAB Function1/1(Euler) -> Gain/1, PID Leader/2(attitude_zyx)
  Constant2/1 -> PID Leader/4(Kp)
  Constant4/1 -> PID Leader/5(Kd)
  Gain/1 -> Scope2/1
  PID Leader/2(angle_error) -> Gain1/1
  Gain2/1 -> Scope4/1
  Attitude Dynamics Leader/2 -> Scope1/1, PID Leader/3(pqr), Mux4/3
  Gain1/1 -> Mux4/2, Scope3/1
  PID Leader/1(Mb) -> Attitude Dynamics Leader/3, Mux4/1, Scope6/1
  Mux4/1 -> To Workspace/1
  theta_cmd/1 -> Mux1/1, PID Leader/1(theta_cmd)
  MATLAB Function1/2(Theta) -> Gain2/1, Mux1/2, Theta Leader/1
  Mux1/1 -> To Workspace1/1

== matlab function system_model_NMPC/Model/control_nmpc/m5 ==
  data: x_f input; P output; rho input
function P = nmpc_parameter_vector(x_f, rho)
% NMPC_PARAMETER_VECTOR
% Creates the parameter vector used by nmpc_orbit_state.
%
% INPUT:
%   x_f(1) = follower semi-major axis, a_f      [m]
%   x_f(2) = follower eccentricity, e_f         [-]
%   x_f(3) = follower inclination, i_f          [rad]
%   x_f(4) = follower argument of periapsis     [rad]
%   x_f(5) = follower RAAN                      [rad]
%   x_f(6) = follower mean anomaly              [rad]
%
%   rho    = atmospheric density                [kg/m^3]
%
% OUTPUT:
%
%   P = [a_f;
%        e_f;
%        i_f;
%        omega_f;
%        rho]

%#codegen

P = zeros(5,1);

P(1) = x_f(1);     % a_f
P(2) = x_f(2);     % e_f
P(3) = x_f(3);     % i_f
P(4) = x_f(4);     % omega_f
P(5) = rho;        % atmospheric density

end

== matlab function system_model_NMPC/Model/Attitude follower /Attitude Leader/MATLAB Function1 ==
  data: quat input; Euler output; Theta output
function [Euler,Theta] = QToTheta(quat)
quat=quat';
Euler = quat2eul( quat );
Theta = Euler(2);
end

== matlab function system_model_NMPC/Model/Attitude follower /Attitude Leader/PID Leader ==
  data: theta_cmd input; Mb output; attitude_zyx input; pqr input; Kp input; Kd input; Mmax input; angle_error output; Mb_raw output
function [Mb, angle_error, Mb_raw] = attitude_pd_controller( ...
    theta_cmd, attitude_zyx, pqr, Kp, Kd, Mmax)
%ATTITUDE_PD_CONTROLLER Spacecraft attitude PD control with torque limits.
%#codegen
%
% Suitable for a Simulink MATLAB Function block. Configure theta_cmd as
% a scalar and all other inputs as fixed-size [3 1] real double vectors.
% All outputs are fixed-size [3 1] column vectors.
%
% INPUTS
%   theta_cmd    Desired pitch [rad]; desired roll and yaw are zero.
%   attitude_zyx Measured ZYX Euler angles [yaw; pitch; roll] [rad].
%   pqr          Body angular rates [p; q; r] [rad/s].
%   Kp           Proportional gains [roll; pitch; yaw] [N*m/rad].
%   Kd           Derivative gains [roll; pitch; yaw] [N*m*s/rad].
%   Mmax         Nonnegative torque limits [roll; pitch; yaw] [N*m].
%
% OUTPUTS (body-axis order: roll/x, pitch/y, yaw/z)
%   Mb           Saturated commanded body torque [N*m].
%   angle_error  Wrapped measured-minus-command Euler errors [rad].
%   Mb_raw       Unsaturated commanded body torque [N*m].
%
% ASSUMPTIONS
%   Inputs are finite; gains and limits are nonnegative. Body rates are
%   measured relative to the attitude reference frame (e.g. LVLH), and
%   desired relative body rates are zero. No command-rate feedforward is
%   included. Body rates are not generally equal to Euler angle rates.
%   This componentwise Euler PD law is intended for operation away from
%   the ZYX Euler singularity at pitch = +/-pi/2; it is not a global
%   attitude controller. Wrapping each error does not remove that
%   singularity.

% Allocate fixed-size column outputs for MATLAB Coder / Simulink.
Mb = zeros(3, 1);
angle_error = zeros(3, 1);
Mb_raw = zeros(3, 1);

% Reorder [yaw; pitch; roll] into body-axis [roll; pitch; yaw],
% then subtract the command [0; theta_cmd; 0]. Explicit indexing
% avoids implicit expansion and preserves fixed-size column handling.
error_unwrapped = zeros(3, 1);
error_unwrapped(1) = attitude_zyx(3);
error_unwrapped(2) = attitude_zyx(2) - theta_cmd;
error_unwrapped(3) = attitude_zyx(1);

for axis = 1:3
    % Wrap measured-minus-command error to [-pi, pi].
    angle_error(axis) = atan2(sin(error_unwrapped(axis)), ...
                             cos(error_unwrapped(axis)));

    % Componentwise equivalent of -Kp.*angle_error - Kd.*pqr.
    Mb_raw(axis) = -Kp(axis) * angle_error(axis) ...
                  -Kd(axis) * pqr(axis);

    % Independently saturate each body torque to +/-Mmax(axis).
    Mb(axis) = min(max(Mb_raw(axis), -Mmax(axis)), Mmax(axis));
end
end

== matlab function system_model_NMPC/Model/Attitude follower /theta cmd Follower ==
  data: beta_c input; theta_rad output
function theta_rad = beta_to_theta(beta_c)
% BETA_TO_THETA  Convert a ballistic coefficient to a pitch angle (rad)
%                using the rising branch of the beta(theta) curve.
%
%   theta_deg = beta_to_theta(beta_c)
%
%   The beta(theta) lookup table is built ONCE (on the first call) and
%   cached in persistent variables. Every subsequent call only does a
%   1-D interpolation, so this is cheap to call repeatedly (e.g. inside
%   a Simulink MATLAB Function block or NMPC cost/constraint function).

    persistent beta_rising theta_rising B_min B_max initialized

    if isempty(initialized)
        [beta_rising, theta_rising, B_min, B_max] = build_beta_theta_table();
        initialized = true;
    end

    if beta_c < B_min || beta_c > B_max
        % Clamp instead of erroring - keeps this safe for Simulink
        % compile-time probing (zero/default inputs) and NMPC solver
        % excursions outside the achievable range.
        beta_c = min(max(beta_c, B_min), B_max);
    end

    theta_rad = interp1(beta_rising, theta_rising, beta_c, 'linear');
    theta_deg = theta_rad * 180/pi;

end


function [beta_rising, theta_rising, B_min, B_max] = build_beta_theta_table()

    n = 4; % power number of data
    num_points = 90*10^n + 1;

    m = 2; % spacecraft mass [kg]

    % C_d model constant (NRLMSISE-00 based)
    alpha = (7.5*10^(-17)*5.14*10^7*10^6*1011) / (1.0 + (7.5*10^(-17)*5.14*10^7*10^6*1011));
    r = sqrt(1-alpha);

    C_d_vec       = zeros(num_points,1);
    theta_vec     = zeros(num_points,1);
    A_ref_tot_vec = zeros(num_points,1);

    for k = 1:num_points

        theta = (pi/(180*10^n))*(k-1); % pitch of satellite [rad]

        % flat plate at incidence theta
        C_d_flat_theta     = 2*(1+(2/3)*r*sin(theta));
        C_d_flat_theta_inv = 2*(1+(2/3)*r*sin(pi/2-theta));

        % Areas
        % 2 solar panels
        A_tot_solar = 2*15*15/10^4;
        A_ref_solar = A_tot_solar*sin(theta);

        % box (front and upper side)
        A_tot_box_front = 10*10/10^4;
        A_tot_box_top   = 15*10/10^4;

        A_ref_box_front = A_tot_box_front*cos(theta);
        A_ref_box_top   = A_tot_box_top*sin(theta);

        A_ref_tot = A_ref_solar + A_ref_box_top + A_ref_box_front;

        % Total drag coefficient (area-weighted blend)
        C_d_total = (A_ref_box_front/A_ref_tot)*C_d_flat_theta_inv ...
                  + ((A_ref_tot-A_ref_box_front)/A_ref_tot)*C_d_flat_theta;

        C_d_vec(k)       = C_d_total;
        theta_vec(k)     = theta;
        A_ref_tot_vec(k) = A_ref_tot;
    end

    beta_vec = (A_ref_tot_vec.*C_d_vec)/m;

    % Restrict to the rising branch only: theta = 0 to peak
    [beta_pk, idx_pk] = max(beta_vec);

    theta_rising = theta_vec(1:idx_pk);
    beta_rising  = beta_vec(1:idx_pk);

    B_min = min(beta_rising);
    B_max = beta_pk;

end

== matlab function system_model_NMPC/Model/Attitude follower /theta cmd Leader ==
  data: beta_c input; theta_rad output
function theta_rad = beta_to_theta(beta_c)
% BETA_TO_THETA  Convert a ballistic coefficient to a pitch angle (deg)
%                using the rising branch of the beta(theta) curve.
%
%   theta_deg = beta_to_theta(beta_c)
%
%   The beta(theta) lookup table is built ONCE (on the first call) and
%   cached in persistent variables. Every subsequent call only does a
%   1-D interpolation, so this is cheap to call repeatedly (e.g. inside
%   a Simulink MATLAB Function block or NMPC cost/constraint function).

    persistent beta_rising theta_rising B_min B_max initialized

    if isempty(initialized)
        [beta_rising, theta_rising, B_min, B_max] = build_beta_theta_table();
        initialized = true;
    end

    if beta_c < B_min || beta_c > B_max
        % Clamp instead of erroring - keeps this safe for Simulink
        % compile-time probing (zero/default inputs) and NMPC solver
        % excursions outside the achievable range.
        beta_c = min(max(beta_c, B_min), B_max);
    end

    theta_rad = interp1(beta_rising, theta_rising, beta_c, 'linear');
    theta_deg = theta_rad * 180/pi;

end


function [beta_rising, theta_rising, B_min, B_max] = build_beta_theta_table()

    n = 4; % power number of data
    num_points = 90*10^n + 1;

    m = 2; % spacecraft mass [kg]

    % C_d model constant (NRLMSISE-00 based)
    alpha = (7.5*10^(-17)*5.14*10^7*10^6*1011) / (1.0 + (7.5*10^(-17)*5.14*10^7*10^6*1011));
    r = sqrt(1-alpha);

    C_d_vec       = zeros(num_points,1);
    theta_vec     = zeros(num_points,1);
    A_ref_tot_vec = zeros(num_points,1);

    for k = 1:num_points

        theta = (pi/(180*10^n))*(k-1); % pitch of satellite [rad]

        % flat plate at incidence theta
        C_d_flat_theta     = 2*(1+(2/3)*r*sin(theta));
        C_d_flat_theta_inv = 2*(1+(2/3)*r*sin(pi/2-theta));

        % Areas
        % 2 solar panels
        A_tot_solar = 2*15*15/10^4;
        A_ref_solar = A_tot_solar*sin(theta);

        % box (front and upper side)
        A_tot_box_front = 10*10/10^4;
        A_tot_box_top   = 15*10/10^4;

        A_ref_box_front = A_tot_box_front*cos(theta);
        A_ref_box_top   = A_tot_box_top*sin(theta);

        A_ref_tot = A_ref_solar + A_ref_box_top + A_ref_box_front;

        % Total drag coefficient (area-weighted blend)
        C_d_total = (A_ref_box_front/A_ref_tot)*C_d_flat_theta_inv ...
                  + ((A_ref_tot-A_ref_box_front)/A_ref_tot)*C_d_flat_theta;

        C_d_vec(k)       = C_d_total;
        theta_vec(k)     = theta;
        A_ref_tot_vec(k) = A_ref_tot;
    end

    beta_vec = (A_ref_tot_vec.*C_d_vec)/m;

    % Restrict to the rising branch only: theta = 0 to peak
    [beta_pk, idx_pk] = max(beta_vec);

    theta_rising = theta_vec(1:idx_pk);
    beta_rising  = beta_vec(1:idx_pk);

    B_min = min(beta_rising);
    B_max = beta_pk;

end

== matlab function system_model_NMPC/Model/orbit_Propegation/Cart2kep Leader ==
  data: r_vec input; a output; v_vec input; mu input; e output; i output; omega output; Omega output; nu output; M output
function [a,e,i,omega,Omega,nu,M] = cart2kep_simulink(r_vec,v_vec,mu)
% CART2KEP_SIMULINK  Simulink/code-generation friendly Cartesian -> Keplerian.
%
% Inputs
%   r_vec : 3-element inertial position vector
%   v_vec : 3-element inertial velocity vector
%   mu    : gravitational parameter
%
% IMPORTANT:
%   Units must be consistent. For the current thesis model use:
%       r_vec [m], v_vec [m/s], mu [m^3/s^2]
%
% Outputs
%   a      semi-major axis
%   e      eccentricity
%   i      inclination [rad]
%   omega  argument of perigee [rad]
%   Omega  RAAN [rad]
%   nu     true anomaly [rad]
%   M      mean anomaly [rad]
%
% Output order is intentionally:
%   [a,e,i,omega,Omega,nu,M]
% so the first six values can be sent directly to osc2mean:
%   [a;e;i;omega;Omega;nu]
%
%#codegen

% -------------------------------------------------------------------------
% Force fixed 1x3 internal vectors WITHOUT r_vec(:)' or variable-size reshape.
% This is friendly to Simulink dimension propagation whether the input port is
% configured as a 3x1 or 1x3 three-element vector.
% -------------------------------------------------------------------------
r3 = [r_vec(1), r_vec(2), r_vec(3)];
v3 = [v_vec(1), v_vec(2), v_vec(3)];

% Magnitudes and radial velocity
rmag = sqrt(r3(1)^2 + r3(2)^2 + r3(3)^2);
v2   = v3(1)^2 + v3(2)^2 + v3(3)^2;

% Specific angular momentum h = r x v
hvec = [ ...
    r3(2)*v3(3) - r3(3)*v3(2), ...
    r3(3)*v3(1) - r3(1)*v3(3), ...
    r3(1)*v3(2) - r3(2)*v3(1)];

hmag = sqrt(hvec(1)^2 + hvec(2)^2 + hvec(3)^2);

% Inclination: atan2 form is numerically safer than acos(hz/h)
i = atan2(sqrt(hvec(1)^2 + hvec(2)^2), hvec(3));

% Node vector n = k x h = [-hy, hx, 0]
nvec = [-hvec(2), hvec(1), 0.0];
nmag = sqrt(nvec(1)^2 + nvec(2)^2);

% Eccentricity vector e = (v x h)/mu - r/|r|
vxh = [ ...
    v3(2)*hvec(3) - v3(3)*hvec(2), ...
    v3(3)*hvec(1) - v3(1)*hvec(3), ...
    v3(1)*hvec(2) - v3(2)*hvec(1)];

evec = vxh/mu - r3/rmag;
e = sqrt(evec(1)^2 + evec(2)^2 + evec(3)^2);

% Semi-major axis from vis-viva
a = 1.0/(2.0/rmag - v2/mu);

% Small tolerance only for singular geometry handling.
% The current thesis baseline (e=0.001, i=20 deg) is far from these limits.
tol = 1.0e-12;

% -------------------------------------------------------------------------
% RAAN
% -------------------------------------------------------------------------
if nmag > tol
    Omega = wrap2pi_local(atan2(nvec(2),nvec(1)));
else
    % Equatorial orbit: RAAN is undefined. Use zero as a nonsingular
    % convention so downstream code receives a finite value.
    Omega = 0.0;
end

% -------------------------------------------------------------------------
% Argument of perigee
% Use atan2(sin,cos) rather than acos + quadrant branching.
% -------------------------------------------------------------------------
if (e > tol) && (nmag > tol)
    c_omega = (nvec(1)*evec(1) + nvec(2)*evec(2) + nvec(3)*evec(3)) ...
              /(nmag*e);

    nxev = [ ...
        nvec(2)*evec(3) - nvec(3)*evec(2), ...
        nvec(3)*evec(1) - nvec(1)*evec(3), ...
        nvec(1)*evec(2) - nvec(2)*evec(1)];

    s_omega = (nxev(1)*hvec(1) + nxev(2)*hvec(2) + nxev(3)*hvec(3)) ...
              /(nmag*e*hmag);

    omega = wrap2pi_local(atan2(s_omega,c_omega));

elseif e > tol
    % Equatorial eccentric orbit: longitude of periapsis is used with
    % Omega = 0, therefore omega carries that angle.
    omega = wrap2pi_local(atan2(evec(2),evec(1)));

else
    % Circular orbit: periapsis direction is undefined.
    omega = 0.0;
end

% -------------------------------------------------------------------------
% True anomaly
% -------------------------------------------------------------------------
if e > tol
    c_nu = (evec(1)*r3(1) + evec(2)*r3(2) + evec(3)*r3(3))/(e*rmag);

    exr = [ ...
        evec(2)*r3(3) - evec(3)*r3(2), ...
        evec(3)*r3(1) - evec(1)*r3(3), ...
        evec(1)*r3(2) - evec(2)*r3(1)];

    s_nu = (exr(1)*hvec(1) + exr(2)*hvec(2) + exr(3)*hvec(3)) ...
           /(e*rmag*hmag);

    nu = wrap2pi_local(atan2(s_nu,c_nu));

elseif nmag > tol
    % Circular inclined orbit: use argument of latitude as nu while omega=0.
    c_u = (nvec(1)*r3(1) + nvec(2)*r3(2) + nvec(3)*r3(3))/(nmag*rmag);

    nxr = [ ...
        nvec(2)*r3(3) - nvec(3)*r3(2), ...
        nvec(3)*r3(1) - nvec(1)*r3(3), ...
        nvec(1)*r3(2) - nvec(2)*r3(1)];

    s_u = (nxr(1)*hvec(1) + nxr(2)*hvec(2) + nxr(3)*hvec(3)) ...
          /(nmag*rmag*hmag);

    nu = wrap2pi_local(atan2(s_u,c_u));

else
    % Circular equatorial orbit: use true longitude as nu.
    nu = wrap2pi_local(atan2(r3(2),r3(1)));
end

% -------------------------------------------------------------------------
% Mean anomaly for elliptic orbit
% For e=0 this correctly reduces to M = nu.
% -------------------------------------------------------------------------
root_term = max(0.0,1.0-e^2);
E = atan2(sqrt(root_term)*sin(nu), e + cos(nu));
E = wrap2pi_local(E);
M = wrap2pi_local(E - e*sin(E));

end


function ang = wrap2pi_local(ang)
% Fixed-scalar wrap into [0,2*pi)
ang = mod(ang,2.0*pi);
if ang < 0.0
    ang = ang + 2.0*pi;
end
end
